simulink model "kanonik"  (R2025b)
settings: Solver=VariableStepAuto  StartTime=0.0  StopTime=10.0  RelTol=1e-3
undefined symbols (not defined in the file): Ac, Ao, Bc, Bo, Cc, Co, Dc, Do
settings Model: Creator=emin  LastModifiedBy=emin

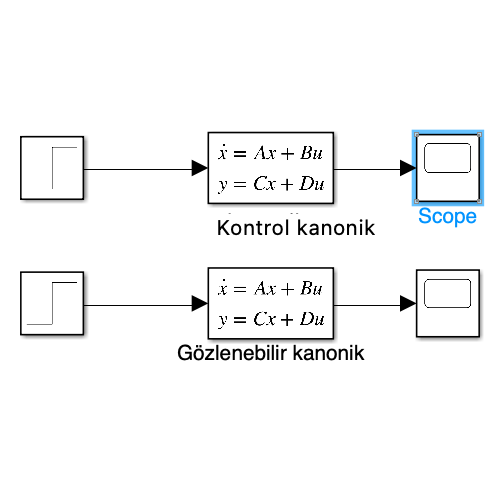
[thumbnail: Simulink's stored preview of the top-level diagram]
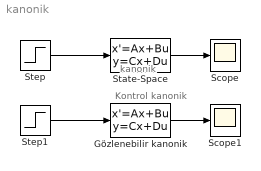
== system kanonik ==
  note: Kontrol kanonik
  note: kanonik
  Gözlenebilir kanonik : StateSpace  A=Ao  B=Bo  C=Co  D=Do  InitialCondition=0
  Scope : Scope
      settings: ActiveDisplayYMinimum=-0.31848608345725249  ActiveDisplayYMaximum=2.8663747511152731
  Scope1 : Scope
      settings: ActiveDisplayYMinimum=-0.31848608345725493  ActiveDisplayYMaximum=2.8663747511152948
  State-Space : StateSpace  A=Ac  B=Bc  C=Cc  D=Dc  InitialCondition=0
  Step : Step  SampleTime=0
  Step1 : Step  SampleTime=0
  wires:
  State-Space/1 -> Scope/1
  Step/1 -> State-Space/1
  Gözlenebilir kanonik/1 -> Scope1/1
  Step1/1 -> Gözlenebilir kanonik/1
